simulink model "E5_nonLinear"  (R2024a)
settings: Solver=VariableStepAuto  StartTime=0.0  StopTime=10.0  RelTol=1e-3
settings Model: Creator=Sanagostar  LastModifiedBy=Sanagostar

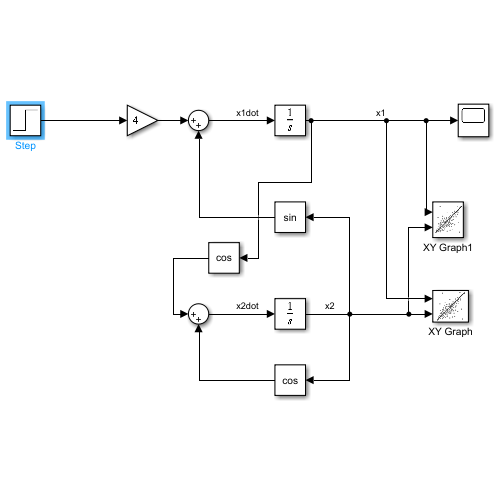
[thumbnail: Simulink's stored preview of the top-level diagram]
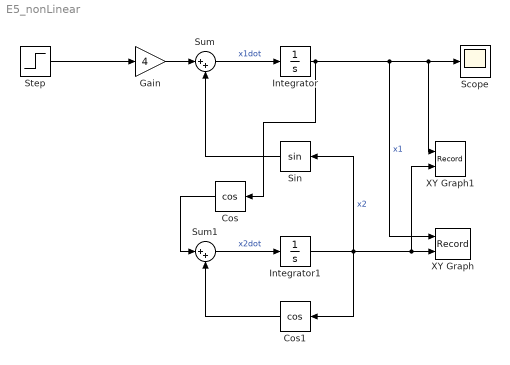
== system E5_nonLinear ==
  Cos : Trigonometry  Operator=cos
  Cos1 : Trigonometry  Operator=cos
  Gain : Gain  Gain=4
  Integrator : Integrator  InitialCondition=5
  Integrator1 : Integrator  InitialCondition=2
  Scope : Scope
  Sin : Trigonometry
  Step : Step  Time=0  SampleTime=0
  Sum : Sum  Inputs=|++
  Sum1 : Sum  Inputs=|++
  XY Graph : Record  FileSettingsInternal="{\"entries\":[{\"content\":{\"excelSettings\":{\"content\":{},\"type\":\"Streamout.ExcelSettings\"}},\"type\":\"Streamout.FileSettingStorage\",\"uuid\":\"\"}],\"packageUris\":[\"http:\\/\\/schema.mathworks.com\\/mf0\\/streamout_blocks\\/R2020a\"],\"version\":\"1.0\"}"  Layout=[1 1]  SignalsInternal="{\"entries\":[{\"content\":{},\"type\":\"RecordBlkView.InputSignals\",\"uuid\":\"\"}],\"packageUris\":[\"http:\\/\\/schema.mathworks.com\\/mf0\\/streamout_blocks\\/R2020a\"],\"version\":\"1.0\"}"  VisualizationBindings="{\"xyplotplugin\":{\"info\":[{\"series\":[],\"subplotID\":1}]}}"  CompatibilityTag=XY
  XY Graph1 : Record  FileSettingsInternal="{\"entries\":[{\"content\":{\"excelSettings\":{\"content\":{},\"type\":\"Streamout.ExcelSettings\"}},\"type\":\"Streamout.FileSettingStorage\",\"uuid\":\"\"}],\"packageUris\":[\"http:\\/\\/schema.mathworks.com\\/mf0\\/streamout_blocks\\/R2020a\"],\"version\":\"1.0\"}"  Layout=[1 1]  SignalsInternal="{\"entries\":[{\"content\":{\"signals\":[{\"content\":{\"blockPath\":[],\"dimensions\":[1],\"domain\":\"\",\"lineColor\":\"#a2142f\",\"port\":1,\"sid\":[\"\"],\"signalID\":1,\"signalName\":\"x1\"},\"type\":\"RecordBlkView.Signal\",\"uuid\":\"\"},{\"content\":{\"blockPath\":[],\"dimensions\":[1],\"domain\":\"\",\"lineColor\":\"#139fff\",\"port\":2,\"sid\":[\"\"],\"signalID\":2,\"signalName\":\"x2\"},\"type\":\"RecordBlkView.Signal\",\"uuid\":\"\"},{\"content\":{\"blockPath\":[],\"dimensions\":[1],\"domain\":\"\",\"lineColor\":\"#a2142f\",\"plots\":[ 1 ],\"port\":1,\"sid\":[\"\"],\"signalID\":3,\"signalName\":\"x1\"},\"type\":\"RecordBlkView.Signal\",\"uuid\":\"\"},{\"content\":{\"blockPath\":[],\"dimensions\":[1],\"domain\":\"\",\"lineColor\":\"#139fff\",\"plots\":[ 1 ],\"port\":2,\"sid\":[\"\"],\"signalID\":4,\"signalName\":\"x2\"},\"type\":\"RecordBlkView.Signal\",\"uuid\":\"\"}]},\"type\":\"RecordBlkView.InputSignals\",\"uuid\":\"\"}],\"packageUris\":[\"http:\\/\\/schema.mathworks.com\\/mf0\\/streamout_blocks\\/R2020a\"],\"version\":\"1.0\"}"  VisualizationBindings="{\"xyplotplugin\":{\"info\":[{\"series\":[{\"bindingParametersList\":[{\"parameter\":\"X-Axis\",\"signalID\":3,\"signalName\":\"x1\"},{\"parameter\":\"Y-Axis\",\"signalID\":4,\"signalName\":\"x2\"}],\"seriesID\":0}],\"subplotID\":1}]}}"  CompatibilityTag=XY  st=-1
  wires:
  Gain/1 -> Sum/1
  Integrator1/1 -> Cos1/1, XY Graph1/2, XY Graph/2, Sin/1  "x2"
  Sin/1 -> Sum/2
  Sum/1 -> Integrator/1  "x1dot"
  Integrator/1 -> XY Graph/1, XY Graph1/1, Scope/1, Cos/1  "x1"
  Sum1/1 -> Integrator1/1  "x2dot"
  Cos/1 -> Sum1/1
  Step/1 -> Gain/1
  Cos1/1 -> Sum1/2
